simulink model "sfLeaveFixed"  (R2025b)
settings: Solver=VariableStepAuto  StartTime=0.0  StopTime=10.0  RelTol=1e-3
settings Model: Creator=The MathWorks, Inc.  LastModifiedBy=The MathWorks, Inc.

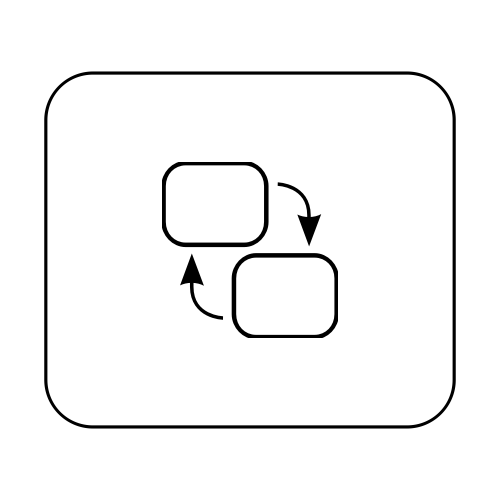
[thumbnail: Simulink's stored preview of the top-level diagram]
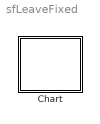
== system sfLeaveFixed ==
  Chart : Stateflow chart  TreatAsAtomicUnit=on

== stateflow chart sfLeaveFixed/Chart ==
  state A
  state B
  (default) -> A
  A -> B : every(5,tick)
  B -> A
